simulink model "ElectricVehicleThermalManagementWithHeatPump"  (R2024b)
settings: Solver=VariableStepAuto  StartTime=0.0  StopTime=3600  RelTol=1e-3  AbsTol=1e-3
PreLoadFcn:
  | init_nmpc
InitFcn:
  | init_nmpc
model workspace: external: MATLAB File ElectricVehicleThermalManagementWithHeatPumpParameters.m (data not in the file)
values from neighbouring files (symbols this model uses):
  battery_C1_LUT = [1913.6 12447 30609 ... (first row only)    [ElectricVehicleThermalManagementWithHeatPumpParameters.m]
  battery_capacity_LUT = [280.081 276.25 276.392]    [ElectricVehicleThermalManagementWithHeatPumpParameters.m]
  battery_cell_cp = 795    [ElectricVehicleThermalManagementWithHeatPumpParameters.m]
  battery_cell_mass = 2.5    [ElectricVehicleThermalManagementWithHeatPumpParameters.m]
  battery_Em_LUT = [3.4966 3.5057 3.5148 ... (first row only)    [ElectricVehicleThermalManagementWithHeatPumpParameters.m]
  battery_N_cells = 20    [ElectricVehicleThermalManagementWithHeatPumpParameters.m]
  battery_Qe_init = 0    [ElectricVehicleThermalManagementWithHeatPumpParameters.m]
  battery_R0_LUT = [0.0117 0.0085 0.009 ... (first row only)    [ElectricVehicleThermalManagementWithHeatPumpParameters.m]
  battery_R1_LUT = [0.0109 0.0029 0.0013 ... (first row only)    [ElectricVehicleThermalManagementWithHeatPumpParameters.m]
  battery_SOC_LUT = [0; 0.1; 0.25; 0.5; 0.75; 0.9; 1]    [ElectricVehicleThermalManagementWithHeatPumpParameters.m]
  battery_T_init = -10    [ElectricVehicleThermalManagementWithHeatPumpParameters.m]
  battery_temperature_LUT = [5 20 40]    [ElectricVehicleThermalManagementWithHeatPumpParameters.m]
  cabin_duct_area = 0.04    [ElectricVehicleThermalManagementWithHeatPumpParameters.m]
  cabin_T_init = -10    [ElectricVehicleThermalManagementWithHeatPumpParameters.m]
  chiller_area_primary = 0.43982297150257105    (= 0.439822971503)    [ElectricVehicleThermalManagementWithHeatPumpParameters.m]
  chiller_N_baffles = 3    [ElectricVehicleThermalManagementWithHeatPumpParameters.m]
  chiller_N_tubes = 100    [ElectricVehicleThermalManagementWithHeatPumpParameters.m]
  chiller_tube_D = 0.0035    [ElectricVehicleThermalManagementWithHeatPumpParameters.m]
  chiller_tube_L = 0.4    [ElectricVehicleThermalManagementWithHeatPumpParameters.m]
  chiller_wall_conductivity = 240    [ElectricVehicleThermalManagementWithHeatPumpParameters.m]
  chiller_wall_thickness = 0.0001    [ElectricVehicleThermalManagementWithHeatPumpParameters.m]
  cond_evap_air_area_flow = 0.3906    [ElectricVehicleThermalManagementWithHeatPumpParameters.m]
  cond_evap_air_area_primary = 1.4834999999999998    (= 1.4835)    [ElectricVehicleThermalManagementWithHeatPumpParameters.m]
  cond_evap_W = 0.015    [ElectricVehicleThermalManagementWithHeatPumpParameters.m]
  cond_evap_wall_conductivity = 240    [ElectricVehicleThermalManagementWithHeatPumpParameters.m]
  cond_evap_wall_thickness = 0.0001    [ElectricVehicleThermalManagementWithHeatPumpParameters.m]
  coolant_channel_D = 0.0092    [ElectricVehicleThermalManagementWithHeatPumpParameters.m]
  coolant_pipe_D = 0.019    [ElectricVehicleThermalManagementWithHeatPumpParameters.m]
  coolant_T_init = -10    [ElectricVehicleThermalManagementWithHeatPumpParameters.m]
  coolant_tank_area = 0.0121    [ElectricVehicleThermalManagementWithHeatPumpParameters.m]
  coolant_tank_volume = 1.25    [ElectricVehicleThermalManagementWithHeatPumpParameters.m]
  coolant_valve_D_ratio_max = 0.95    [ElectricVehicleThermalManagementWithHeatPumpParameters.m]
  coolant_valve_D_ratio_min = 0.001    [ElectricVehicleThermalManagementWithHeatPumpParameters.m]
  coolant_valve_displacement = 0.0063    [ElectricVehicleThermalManagementWithHeatPumpParameters.m]
  coolant_valve_S_max = 0.0053    [ElectricVehicleThermalManagementWithHeatPumpParameters.m]
  evaporator_air_area_flow = 0.12    [ElectricVehicleThermalManagementWithHeatPumpParameters.m]
  evaporator_air_area_primary = 0.4323    [ElectricVehicleThermalManagementWithHeatPumpParameters.m]
  evaporator_W = 0.015    [ElectricVehicleThermalManagementWithHeatPumpParameters.m]
  evaporator_wall_conductivity = 240    [ElectricVehicleThermalManagementWithHeatPumpParameters.m]
  evaporator_wall_thickness = 0.0001    [ElectricVehicleThermalManagementWithHeatPumpParameters.m]
  expansion_valve_D_ratio_max = 0.9    [ElectricVehicleThermalManagementWithHeatPumpParameters.m]
  hex_area_primary = 0.070371675440411369    (= 0.0703716754404)    [ElectricVehicleThermalManagementWithHeatPumpParameters.m]
  hex_N_tubes = 64    [ElectricVehicleThermalManagementWithHeatPumpParameters.m]
  hex_tube_D = 0.0035    [ElectricVehicleThermalManagementWithHeatPumpParameters.m]
  hex_wall_conductivity = 240    [ElectricVehicleThermalManagementWithHeatPumpParameters.m]
  hex_wall_thickness = 0.0001    [ElectricVehicleThermalManagementWithHeatPumpParameters.m]
  inner_cond_air_area_flow = 0.1953    [ElectricVehicleThermalManagementWithHeatPumpParameters.m]
  inner_cond_air_area_primary = 0.99520000000000008    (= 0.9952)    [ElectricVehicleThermalManagementWithHeatPumpParameters.m]
  inner_cond_W = 0.02    [ElectricVehicleThermalManagementWithHeatPumpParameters.m]
  inner_cond_wall_conductivity = 240    [ElectricVehicleThermalManagementWithHeatPumpParameters.m]
  inner_cond_wall_thickness = 0.0001    [ElectricVehicleThermalManagementWithHeatPumpParameters.m]
  pump_speed_max = 1000    [ElectricVehicleThermalManagementWithHeatPumpParameters.m]
  radiator_air_area_flow = 0.097499999999999989    (= 0.0975)    [ElectricVehicleThermalManagementWithHeatPumpParameters.m]
  radiator_air_area_primary = 0.43687499999999996    (= 0.436875)    [ElectricVehicleThermalManagementWithHeatPumpParameters.m]
  radiator_W = 0.015    [ElectricVehicleThermalManagementWithHeatPumpParameters.m]
  radiator_wall_conductivity = 240    [ElectricVehicleThermalManagementWithHeatPumpParameters.m]
  radiator_wall_thickness = 0.0001    [ElectricVehicleThermalManagementWithHeatPumpParameters.m]
  refrigerant_p_init = 0.2    [ElectricVehicleThermalManagementWithHeatPumpParameters.m]
  refrigerant_pipe_D = 0.01    [ElectricVehicleThermalManagementWithHeatPumpParameters.m]
  refrigerant_valve_D_ratio_max = 0.95    [ElectricVehicleThermalManagementWithHeatPumpParameters.m]
  refrigerant_valve_displacement = 0.005    [ElectricVehicleThermalManagementWithHeatPumpParameters.m]
libraries: fl_lib x227, nesl_utility x162, SimscapeFluids_lib x30, LiBatteryElements_lib x16, slpidlib x3, SignalEditorBlockLib x1
(part 12 of 13)

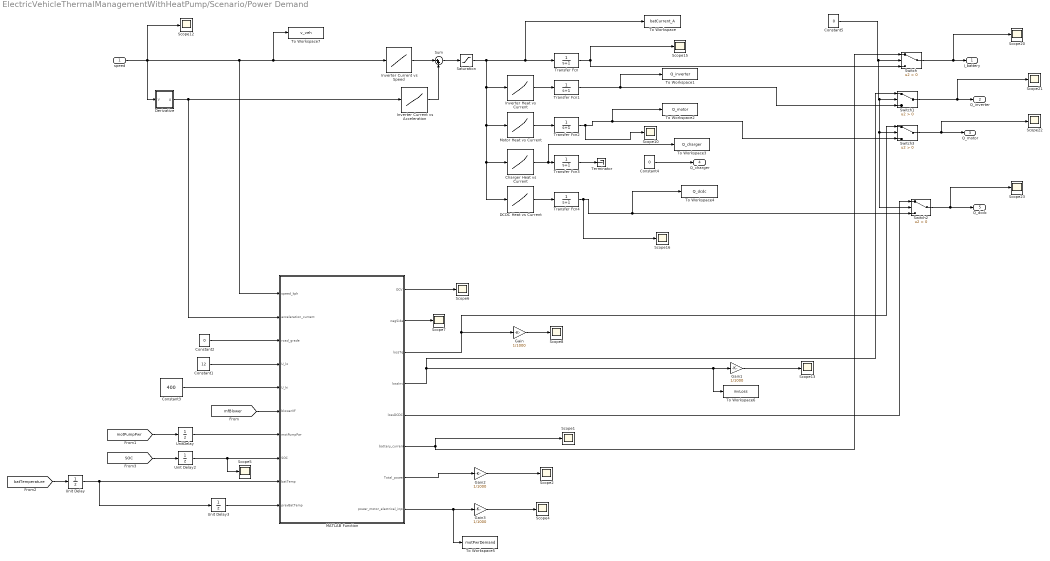
== system ElectricVehicleThermalManagementWithHeatPump/Scenario/Power Demand ==
  speed : Inport
  Charger Heat vs Current : Lookup_n-D  NumberOfTableDimensions=1  BreakpointsForDimension1=[-100 0 25 50 300]  IndexSearchMethod=Linear search  BeginIndexSearchUsingPreviousIndexResult=on  Table=[250 0 40 70 400]  InternalRulePriority=Speed  RndMeth=Simplest
  Constant1 : Constant  Value=12
  Constant2 : Constant  Value=0
  Constant3 : Constant  Value=400
  Constant4 : Constant  Value=0
  Constant5 : Constant  Value=0
  DCDC Heat vs Current : Lookup_n-D  NumberOfTableDimensions=1  BreakpointsForDimension1=[-100 0 25 50 300]  IndexSearchMethod=Linear search  BeginIndexSearchUsingPreviousIndexResult=on  Table=[250 0 40 70 400]  InternalRulePriority=Speed  RndMeth=Simplest
  Derivative : Subsystem  mask(1-st Order Filter Derivative){tau=1}
      mask prompts: tau "Filter time constant [s]"
  Gain{,1..3} (4 alike) : Gain  Gain=1/1000
  Inverter Current vs Acceleration : Lookup_n-D  NumberOfTableDimensions=1  BreakpointsForDimension1=[-10 -8 -5 0 5 8 10]  IndexSearchMethod=Linear search  BeginIndexSearchUsingPreviousIndexResult=on  Table=[200 150 100 0 100 150 200]*0.6  InternalRulePriority=Speed  RndMeth=Simplest
  Inverter Current vs Speed : Lookup_n-D  NumberOfTableDimensions=1  BreakpointsForDimension1=[0 60 80 100 120 140 160 180 200]  IndexSearchMethod=Linear search  BeginIndexSearchUsingPreviousIndexResult=on  Table=[0 10 18 27 45 65 100 120 160]  InternalRulePriority=Speed  RndMeth=Simplest
  Inverter Heat vs Current : Lookup_n-D  NumberOfTableDimensions=1  BreakpointsForDimension1=[-100 0 25 50 300]  IndexSearchMethod=Linear search  BeginIndexSearchUsingPreviousIndexResult=on  Table=[250 0 40 70 400]  InternalRulePriority=Speed  RndMeth=Simplest
  MATLAB Function : MATLAB Function  TreatAsAtomicUnit=on
  Motor Heat vs Current : Lookup_n-D  NumberOfTableDimensions=1  BreakpointsForDimension1=[-150 -70 -26 0 25 50 100 300 600]  IndexSearchMethod=Linear search  BeginIndexSearchUsingPreviousIndexResult=on  Table=[3500 2650 2100 0 400 550 4800 4800 4800]  InternalRulePriority=Speed  RndMeth=Simplest
  Saturation : Saturate  UpperLimit=200  LowerLimit=-inf  ZeroCross=off
  Scope{1..2,4..8,10,12..13,15..16,20..23} (16 alike) : Scope
  Sum : Sum  Inputs=|++
  Switch{,1..3} (4 alike) : Switch  Criteria=u2 > Threshold  SaturateOnIntegerOverflow=off  InputSameDT=off
  Terminator : Terminator
  To Workspace : ToWorkspace  VariableName=batCurrent_A  SampleTime=-1
  To Workspace1 : ToWorkspace  VariableName=Q_inverter  SampleTime=-1
  To Workspace2 : ToWorkspace  VariableName=Q_motor  SampleTime=-1
  To Workspace3 : ToWorkspace  VariableName=Q_charger  SampleTime=-1
  To Workspace4 : ToWorkspace  VariableName=Q_dcdc  SampleTime=-1
  To Workspace5 : ToWorkspace  VariableName=motPwrDemand  SampleTime=-1
  To Workspace6 : ToWorkspace  VariableName=invLoss  SampleTime=-1
  To Workspace7 : ToWorkspace  VariableName=v_veh  SampleTime=-1
  Transfer Fcn{,1..4} (5 alike) : TransferFcn  Denominator=[1 1]
  Unit Delay : UnitDelay  SampleTime=-1  HasFrameUpgradeWarning=on
  Unit Delay2 : UnitDelay  SampleTime=-1  HasFrameUpgradeWarning=on
  Unit Delay3 : UnitDelay  SampleTime=-1  HasFrameUpgradeWarning=on
  UnitDelay : UnitDelay  SampleTime=-1  HasFrameUpgradeWarning=on
  I_battery : Outport
  Q_inverter : Outport  Port=2
  Q_motor : Outport  Port=3
  Q_charger : Outport  Port=4
  Q_dcdc : Outport  Port=5
  wires:
  Derivative/1(A) -> Inverter Current vs Acceleration/1, MATLAB Function/2(acceleration_current)
  speed/1 -> Scope12/1, MATLAB Function/1(speed_kph), To Workspace7/1, Inverter Current vs Speed/1, Derivative/1(V)
  Inverter Current vs Speed/1 -> Sum/1
  Inverter Current vs Acceleration/1 -> Sum/2
  Sum/1 -> Saturation/1
  Inverter Heat vs Current/1 -> Transfer Fcn1/1
  Motor Heat vs Current/1 -> Transfer Fcn2/1
  Charger Heat vs Current/1 -> To Workspace3/1, Transfer Fcn3/1
  Transfer Fcn/1 -> Switch/3, Scope15/1
  Transfer Fcn1/1 -> To Workspace1/1, Switch1/3
  Transfer Fcn2/1 -> Scope10/1, To Workspace2/1, Switch3/3
  DCDC Heat vs Current/1 -> Transfer Fcn4/1
  Transfer Fcn4/1 -> Scope16/1, To Workspace4/1, Switch2/3
  Constant2/1 -> MATLAB Function/3(road_grade)
  MATLAB Function/3(lossTq) -> Switch3/1, Gain/1
  Gain/1 -> Scope8/1
  MATLAB Function/4(lossInv) -> Switch1/1, Gain1/1, To Workspace6/1
  Gain1/1 -> Scope13/1
  MATLAB Function/7(Total_power) -> Gain2/1
  Gain2/1 -> Scope2/1
  Constant1/1 -> MATLAB Function/4(U_lo)
  MATLAB Function/8(power_motor_electrical_input) -> To Workspace5/1, Gain3/1
  Constant3/1 -> MATLAB Function/5(U_hi)
  [mfBlower] -> MATLAB Function/6(blowerVF)
  [batTemperature] -> Unit Delay/1
  [SOC] -> Unit Delay2/1
  Gain3/1 -> Scope4/1
  Saturation/1 -> Inverter Heat vs Current/1, Motor Heat vs Current/1, DCDC Heat vs Current/1, Charger Heat vs Current/1, To Workspace/1, Transfer Fcn/1
  MATLAB Function/6(battery_current) -> Switch/1, Scope1/1
  Switch1/1 -> Scope21/1, Q_inverter/1
  Constant4/1 -> Q_charger/1
  Switch2/1 -> Scope23/1, Q_dcdc/1
  MATLAB Function/5(lossDCDC) -> Switch2/1
  Switch3/1 -> Scope22/1, Q_motor/1
  Constant5/1 -> Switch2/2, Switch3/2, Switch1/2, Switch/2
  Switch/1 -> Scope20/1, I_battery/1
  MATLAB Function/1(OCV) -> Scope6/1
  MATLAB Function/2(negSide) -> Scope7/1
  [motPumpPwr] -> UnitDelay/1
  Unit Delay/1 -> Unit Delay3/1, MATLAB Function/9(batTemp)
  UnitDelay/1 -> MATLAB Function/7(motPumpPwr)
  Unit Delay2/1 -> Scope5/1, MATLAB Function/8(SOC)
  Unit Delay3/1 -> MATLAB Function/10(prevBatTemp)
  Transfer Fcn3/1 -> Terminator/1

== system ElectricVehicleThermalManagementWithHeatPump/Battery/Pack 1/Lithium Cell 1RC ==
  note: Power
      | Losses
  C1 : LiBatteryElements_lib/C_table  C_Table=C1_LUT F  SOC_Table=SOC_LUT  Temp_Table=Temperature_LUT K  v0=0 V
      settings: InternalSimscapePortConfiguration="{\"Bottom\":[],\"Left\":[{\"id\":\"p\",\"label\":\"+\",\"type\":\"foundation.electrical.electrical\"},{\"id\":\"T\",\"label\":\"T\",\"type\":\"input\"},{\"id\":\"SOC\",\"label\":\"SOC\",\"type\":\"input\"}],\"Right\":[{\"id\":\"n\",\"label\":\"-\",\"type\":\"foundation.electrical.electrical\"}],\"Top\":[]}"
  Em_table : LiBatteryElements_lib/Em_table  C_Table=Capacity_LUT hr*A  Em_Table=Em_LUT V  SOC_Table=SOC_LUT  Temp_Table=Temperature_LUT K  Qinit=Qe_init hr*A
      settings: InternalSimscapePortConfiguration="{\"Bottom\":[],\"Left\":[{\"id\":\"p\",\"label\":\"+\",\"type\":\"foundation.electrical.electrical\"},{\"id\":\"C\",\"label\":\"C\",\"type\":\"output\"},{\"id\":\"SOC\",\"label\":\"SOC\",\"type\":\"output\"}],\"Right\":[{\"id\":\"n\",\"label\":\"-\",\"type\":\"foundation.electrical.electrical\"},{\"id\":\"T\",\"label\":\"T\",\"type\":\"input\"}],\"Top\":[]}"
  PS-Simulink Converter : nesl_utility/PS-Simulink Converter  PhysicalDomain=network_engine_domain  SubClassName=ps_output  LeftPortType=input  RightPortType=output  PseudoPeriodic=off  Frequencies=[]  VectorFormat=inherit  Unit=inherit  AffineConversion=off
  PS-Simulink Converter1 : nesl_utility/PS-Simulink Converter  PhysicalDomain=network_engine_domain  SubClassName=ps_output  LeftPortType=input  RightPortType=output  PseudoPeriodic=off  Frequencies=[]  VectorFormat=inherit  Unit=inherit  AffineConversion=off
  Power Sum : fl_lib/Physical Signals/Functions/PS Add
  R0 : LiBatteryElements_lib/R_table  R_Table=R0_LUT Ohm  SOC_Table=SOC_LUT  Temp_Table=Temperature_LUT K
      settings: InternalSimscapePortConfiguration="{\"Bottom\":[],\"Left\":[{\"id\":\"p\",\"label\":\"+\",\"type\":\"foundation.electrical.electrical\"},{\"id\":\"T\",\"label\":\"T\",\"type\":\"input\"},{\"id\":\"SOC\",\"label\":\"SOC\",\"type\":\"input\"}],\"Right\":[{\"id\":\"n\",\"label\":\"-\",\"type\":\"foundation.electrical.electrical\"},{\"id\":\"pow\",\"label\":\"POW\",\"type\":\"output\"}],\"Top\":[]}"
  R1 : LiBatteryElements_lib/R_table  R_Table=R1_LUT Ohm  SOC_Table=SOC_LUT  Temp_Table=Temperature_LUT K
      settings: InternalSimscapePortConfiguration="{\"Bottom\":[],\"Left\":[{\"id\":\"p\",\"label\":\"+\",\"type\":\"foundation.electrical.electrical\"},{\"id\":\"T\",\"label\":\"T\",\"type\":\"input\"},{\"id\":\"SOC\",\"label\":\"SOC\",\"type\":\"input\"}],\"Right\":[{\"id\":\"n\",\"label\":\"-\",\"type\":\"foundation.electrical.electrical\"},{\"id\":\"pow\",\"label\":\"POW\",\"type\":\"output\"}],\"Top\":[]}"
  Scope : Scope
  Scope1 : Scope
  To Workspace : ToWorkspace  VariableName=soc_meas  SampleTime=-1
  P : PMIOPort  Side=Left
  + : PMIOPort  Port=2  Side=Left
  T : PMIOPort  Port=3  Side=Right
  - : PMIOPort  Port=4  Side=Right
  tag scope: SOC=global
  wires:
  PS-Simulink Converter/1 -> To Workspace/1, [SOC], Scope/1
  PS-Simulink Converter1/1 -> Scope1/1
  connections:
  R1/RConn2 -- Power Sum/LConn1
  Power Sum/LConn2 -- R0/RConn2
  P/RConn1 -- Power Sum/RConn1
  +/RConn1 -- R0/RConn1
  T/RConn1 -- Em_table/RConn2 -- R0/LConn2 -- C1/LConn2 -- R1/LConn2
  Em_table/LConn1 -- C1/LConn1 -- R1/LConn1
  C1/RConn1 -- R1/RConn1 -- R0/LConn1
  Em_table/RConn1 -- -/RConn1
  C1/LConn3 -- PS-Simulink Converter/LConn1 -- R0/LConn3 -- Em_table/LConn3 -- R1/LConn3
  PS-Simulink Converter1/LConn1 -- Em_table/LConn2

== system ElectricVehicleThermalManagementWithHeatPump/Battery/Pack 1/Thermal Model ==
  Battery Thermal Mass : fl_lib/Thermal/Thermal Elements/Thermal Mass  mass_type=foundation.enum.constant_variable.constant  mass=cell_mass*Ncells kg  sp_heat=cell_Cp_heat J/kg/K  mass_min=1e-6 kg  num_ports=foundation.enum.numPorts2.one  m_specify=off  m_priority=High  m=1 kg  m_nominal_specify=off  m_nominal_value=1  m_nominal_unit=kg  T_specify=on  T_priority=High  T=T_init K  T_nominal_specify=off  T_nominal_value=1  T_nominal_unit=K  Q_specify=off  Q_priority=None  Q=0 W  Q_nominal_specify=off  Q_nominal_value=1  Q_nominal_unit=W
  Controlled Heat Flow Rate Source : fl_lib/Thermal/Thermal Sources/Controlled Heat Flow Rate Source
  Temperature Sensor : fl_lib/Thermal/Thermal Sensors/Temperature Sensor  temperature_measure=foundation.enum.MeasurementReference.difference
  Thermal Reference : fl_lib/Thermal/Thermal Elements/Thermal Reference
  Thermal Reference2 : fl_lib/Thermal/Thermal Elements/Thermal Reference
  H : PMIOPort  Side=Left
  Pxn : PMIOPort  Port=2  Side=Left
  T : PMIOPort  Port=3  Side=Right
  connections:
  H/RConn1 -- Controlled Heat Flow Rate Source/LConn1 -- Battery Thermal Mass/LConn1 -- Temperature Sensor/LConn1
  Pxn/RConn1 -- Controlled Heat Flow Rate Source/RConn1
  Controlled Heat Flow Rate Source/RConn2 -- Thermal Reference2/LConn1
  Thermal Reference/LConn1 -- Temperature Sensor/RConn1
  T/RConn1 -- Temperature Sensor/RConn2

== system ElectricVehicleThermalManagementWithHeatPump/Battery/Pack 2/Lithium Cell 1RC ==
  note: Power
      | Losses
  C1 : LiBatteryElements_lib/C_table  C_Table=C1_LUT F  SOC_Table=SOC_LUT  Temp_Table=Temperature_LUT K  v0=0 V
      settings: InternalSimscapePortConfiguration="{\"Bottom\":[],\"Left\":[{\"id\":\"p\",\"label\":\"+\",\"type\":\"foundation.electrical.electrical\"},{\"id\":\"T\",\"label\":\"T\",\"type\":\"input\"},{\"id\":\"SOC\",\"label\":\"SOC\",\"type\":\"input\"}],\"Right\":[{\"id\":\"n\",\"label\":\"-\",\"type\":\"foundation.electrical.electrical\"}],\"Top\":[]}"
  Em_table : LiBatteryElements_lib/Em_table  C_Table=Capacity_LUT hr*A  Em_Table=Em_LUT V  SOC_Table=SOC_LUT  Temp_Table=Temperature_LUT K  Qinit=Qe_init hr*A
      settings: InternalSimscapePortConfiguration="{\"Bottom\":[],\"Left\":[{\"id\":\"p\",\"label\":\"+\",\"type\":\"foundation.electrical.electrical\"},{\"id\":\"C\",\"label\":\"C\",\"type\":\"output\"},{\"id\":\"SOC\",\"label\":\"SOC\",\"type\":\"output\"}],\"Right\":[{\"id\":\"n\",\"label\":\"-\",\"type\":\"foundation.electrical.electrical\"},{\"id\":\"T\",\"label\":\"T\",\"type\":\"input\"}],\"Top\":[]}"
  Power Sum : fl_lib/Physical Signals/Functions/PS Add
  R0 : LiBatteryElements_lib/R_table  R_Table=R0_LUT Ohm  SOC_Table=SOC_LUT  Temp_Table=Temperature_LUT K
      settings: InternalSimscapePortConfiguration="{\"Bottom\":[],\"Left\":[{\"id\":\"p\",\"label\":\"+\",\"type\":\"foundation.electrical.electrical\"},{\"id\":\"T\",\"label\":\"T\",\"type\":\"input\"},{\"id\":\"SOC\",\"label\":\"SOC\",\"type\":\"input\"}],\"Right\":[{\"id\":\"n\",\"label\":\"-\",\"type\":\"foundation.electrical.electrical\"},{\"id\":\"pow\",\"label\":\"POW\",\"type\":\"output\"}],\"Top\":[]}"
  R1 : LiBatteryElements_lib/R_table  R_Table=R1_LUT Ohm  SOC_Table=SOC_LUT  Temp_Table=Temperature_LUT K
      settings: InternalSimscapePortConfiguration="{\"Bottom\":[],\"Left\":[{\"id\":\"p\",\"label\":\"+\",\"type\":\"foundation.electrical.electrical\"},{\"id\":\"T\",\"label\":\"T\",\"type\":\"input\"},{\"id\":\"SOC\",\"label\":\"SOC\",\"type\":\"input\"}],\"Right\":[{\"id\":\"n\",\"label\":\"-\",\"type\":\"foundation.electrical.electrical\"},{\"id\":\"pow\",\"label\":\"POW\",\"type\":\"output\"}],\"Top\":[]}"
  P : PMIOPort  Side=Left
  + : PMIOPort  Port=2  Side=Left
  T : PMIOPort  Port=3  Side=Right
  - : PMIOPort  Port=4  Side=Right
  connections:
  R1/RConn2 -- Power Sum/LConn1
  Power Sum/LConn2 -- R0/RConn2
  P/RConn1 -- Power Sum/RConn1
  +/RConn1 -- R0/RConn1
  T/RConn1 -- Em_table/RConn2 -- R0/LConn2 -- C1/LConn2 -- R1/LConn2
  Em_table/LConn1 -- C1/LConn1 -- R1/LConn1
  C1/RConn1 -- R1/RConn1 -- R0/LConn1
  Em_table/RConn1 -- -/RConn1
  C1/LConn3 -- Em_table/LConn3 -- R1/LConn3 -- R0/LConn3

== system ElectricVehicleThermalManagementWithHeatPump/Battery/Pack 2/Thermal Model ==
  Battery Thermal Mass : fl_lib/Thermal/Thermal Elements/Thermal Mass  mass_type=foundation.enum.constant_variable.constant  mass=cell_mass*Ncells kg  sp_heat=cell_Cp_heat J/kg/K  mass_min=1e-6 kg  num_ports=foundation.enum.numPorts2.one  m_specify=off  m_priority=High  m=1 kg  m_nominal_specify=off  m_nominal_value=1  m_nominal_unit=kg  T_specify=on  T_priority=High  T=T_init K  T_nominal_specify=off  T_nominal_value=1  T_nominal_unit=K  Q_specify=off  Q_priority=None  Q=0 W  Q_nominal_specify=off  Q_nominal_value=1  Q_nominal_unit=W
  Controlled Heat Flow Rate Source : fl_lib/Thermal/Thermal Sources/Controlled Heat Flow Rate Source
  Temperature Sensor : fl_lib/Thermal/Thermal Sensors/Temperature Sensor  temperature_measure=foundation.enum.MeasurementReference.difference
  Thermal Reference : fl_lib/Thermal/Thermal Elements/Thermal Reference
  Thermal Reference2 : fl_lib/Thermal/Thermal Elements/Thermal Reference
  H : PMIOPort  Side=Left
  Pxn : PMIOPort  Port=2  Side=Left
  T : PMIOPort  Port=3  Side=Right
  connections:
  H/RConn1 -- Controlled Heat Flow Rate Source/LConn1 -- Battery Thermal Mass/LConn1 -- Temperature Sensor/LConn1
  Pxn/RConn1 -- Controlled Heat Flow Rate Source/RConn1
  Controlled Heat Flow Rate Source/RConn2 -- Thermal Reference2/LConn1
  Thermal Reference/LConn1 -- Temperature Sensor/RConn1
  T/RConn1 -- Temperature Sensor/RConn2

== system ElectricVehicleThermalManagementWithHeatPump/Battery/Pack 3/Lithium Cell 1RC ==
  note: Power
      | Losses
  C1 : LiBatteryElements_lib/C_table  C_Table=C1_LUT F  SOC_Table=SOC_LUT  Temp_Table=Temperature_LUT K  v0=0 V
      settings: InternalSimscapePortConfiguration="{\"Bottom\":[],\"Left\":[{\"id\":\"p\",\"label\":\"+\",\"type\":\"foundation.electrical.electrical\"},{\"id\":\"T\",\"label\":\"T\",\"type\":\"input\"},{\"id\":\"SOC\",\"label\":\"SOC\",\"type\":\"input\"}],\"Right\":[{\"id\":\"n\",\"label\":\"-\",\"type\":\"foundation.electrical.electrical\"}],\"Top\":[]}"
  Em_table : LiBatteryElements_lib/Em_table  C_Table=Capacity_LUT hr*A  Em_Table=Em_LUT V  SOC_Table=SOC_LUT  Temp_Table=Temperature_LUT K  Qinit=Qe_init hr*A
      settings: InternalSimscapePortConfiguration="{\"Bottom\":[],\"Left\":[{\"id\":\"p\",\"label\":\"+\",\"type\":\"foundation.electrical.electrical\"},{\"id\":\"C\",\"label\":\"C\",\"type\":\"output\"},{\"id\":\"SOC\",\"label\":\"SOC\",\"type\":\"output\"}],\"Right\":[{\"id\":\"n\",\"label\":\"-\",\"type\":\"foundation.electrical.electrical\"},{\"id\":\"T\",\"label\":\"T\",\"type\":\"input\"}],\"Top\":[]}"
  Power Sum : fl_lib/Physical Signals/Functions/PS Add
  R0 : LiBatteryElements_lib/R_table  R_Table=R0_LUT Ohm  SOC_Table=SOC_LUT  Temp_Table=Temperature_LUT K
      settings: InternalSimscapePortConfiguration="{\"Bottom\":[],\"Left\":[{\"id\":\"p\",\"label\":\"+\",\"type\":\"foundation.electrical.electrical\"},{\"id\":\"T\",\"label\":\"T\",\"type\":\"input\"},{\"id\":\"SOC\",\"label\":\"SOC\",\"type\":\"input\"}],\"Right\":[{\"id\":\"n\",\"label\":\"-\",\"type\":\"foundation.electrical.electrical\"},{\"id\":\"pow\",\"label\":\"POW\",\"type\":\"output\"}],\"Top\":[]}"
  R1 : LiBatteryElements_lib/R_table  R_Table=R1_LUT Ohm  SOC_Table=SOC_LUT  Temp_Table=Temperature_LUT K
      settings: InternalSimscapePortConfiguration="{\"Bottom\":[],\"Left\":[{\"id\":\"p\",\"label\":\"+\",\"type\":\"foundation.electrical.electrical\"},{\"id\":\"T\",\"label\":\"T\",\"type\":\"input\"},{\"id\":\"SOC\",\"label\":\"SOC\",\"type\":\"input\"}],\"Right\":[{\"id\":\"n\",\"label\":\"-\",\"type\":\"foundation.electrical.electrical\"},{\"id\":\"pow\",\"label\":\"POW\",\"type\":\"output\"}],\"Top\":[]}"
  P : PMIOPort  Side=Left
  + : PMIOPort  Port=2  Side=Left
  T : PMIOPort  Port=3  Side=Right
  - : PMIOPort  Port=4  Side=Right
  connections:
  R0/LConn3 -- R1/LConn3 -- Em_table/LConn3 -- C1/LConn3
  Em_table/RConn1 -- -/RConn1
  R0/LConn1 -- R1/RConn1 -- C1/RConn1
  R1/LConn1 -- C1/LConn1 -- Em_table/LConn1
  R1/LConn2 -- C1/LConn2 -- R0/LConn2 -- Em_table/RConn2 -- T/RConn1
  +/RConn1 -- R0/RConn1
  P/RConn1 -- Power Sum/RConn1
  Power Sum/LConn2 -- R0/RConn2
  R1/RConn2 -- Power Sum/LConn1

== system ElectricVehicleThermalManagementWithHeatPump/Battery/Pack 3/Thermal Model ==
  Battery Thermal Mass : fl_lib/Thermal/Thermal Elements/Thermal Mass  mass_type=foundation.enum.constant_variable.constant  mass=cell_mass*Ncells kg  sp_heat=cell_Cp_heat J/kg/K  mass_min=1e-6 kg  num_ports=foundation.enum.numPorts2.one  m_specify=off  m_priority=High  m=1 kg  m_nominal_specify=off  m_nominal_value=1  m_nominal_unit=kg  T_specify=on  T_priority=High  T=T_init K  T_nominal_specify=off  T_nominal_value=1  T_nominal_unit=K  Q_specify=off  Q_priority=None  Q=0 W  Q_nominal_specify=off  Q_nominal_value=1  Q_nominal_unit=W
  Controlled Heat Flow Rate Source : fl_lib/Thermal/Thermal Sources/Controlled Heat Flow Rate Source
  Temperature Sensor : fl_lib/Thermal/Thermal Sensors/Temperature Sensor  temperature_measure=foundation.enum.MeasurementReference.difference
  Thermal Reference : fl_lib/Thermal/Thermal Elements/Thermal Reference
  Thermal Reference2 : fl_lib/Thermal/Thermal Elements/Thermal Reference
  H : PMIOPort  Side=Left
  Pxn : PMIOPort  Port=2  Side=Left
  T : PMIOPort  Port=3  Side=Right
  connections:
  T/RConn1 -- Temperature Sensor/RConn2
  Thermal Reference/LConn1 -- Temperature Sensor/RConn1
  Controlled Heat Flow Rate Source/RConn2 -- Thermal Reference2/LConn1
  Pxn/RConn1 -- Controlled Heat Flow Rate Source/RConn1
  Temperature Sensor/LConn1 -- Battery Thermal Mass/LConn1 -- Controlled Heat Flow Rate Source/LConn1 -- H/RConn1

== system ElectricVehicleThermalManagementWithHeatPump/Battery/Pack 4/Lithium Cell 1RC ==
  note: Power
      | Losses
  C1 : LiBatteryElements_lib/C_table  C_Table=C1_LUT F  SOC_Table=SOC_LUT  Temp_Table=Temperature_LUT K  v0=0 V
      settings: InternalSimscapePortConfiguration="{\"Bottom\":[],\"Left\":[{\"id\":\"p\",\"label\":\"+\",\"type\":\"foundation.electrical.electrical\"},{\"id\":\"T\",\"label\":\"T\",\"type\":\"input\"},{\"id\":\"SOC\",\"label\":\"SOC\",\"type\":\"input\"}],\"Right\":[{\"id\":\"n\",\"label\":\"-\",\"type\":\"foundation.electrical.electrical\"}],\"Top\":[]}"
  Em_table : LiBatteryElements_lib/Em_table  C_Table=Capacity_LUT hr*A  Em_Table=Em_LUT V  SOC_Table=SOC_LUT  Temp_Table=Temperature_LUT K  Qinit=Qe_init hr*A
      settings: InternalSimscapePortConfiguration="{\"Bottom\":[],\"Left\":[{\"id\":\"p\",\"label\":\"+\",\"type\":\"foundation.electrical.electrical\"},{\"id\":\"C\",\"label\":\"C\",\"type\":\"output\"},{\"id\":\"SOC\",\"label\":\"SOC\",\"type\":\"output\"}],\"Right\":[{\"id\":\"n\",\"label\":\"-\",\"type\":\"foundation.electrical.electrical\"},{\"id\":\"T\",\"label\":\"T\",\"type\":\"input\"}],\"Top\":[]}"
  Power Sum : fl_lib/Physical Signals/Functions/PS Add
  R0 : LiBatteryElements_lib/R_table  R_Table=R0_LUT Ohm  SOC_Table=SOC_LUT  Temp_Table=Temperature_LUT K
      settings: InternalSimscapePortConfiguration="{\"Bottom\":[],\"Left\":[{\"id\":\"p\",\"label\":\"+\",\"type\":\"foundation.electrical.electrical\"},{\"id\":\"T\",\"label\":\"T\",\"type\":\"input\"},{\"id\":\"SOC\",\"label\":\"SOC\",\"type\":\"input\"}],\"Right\":[{\"id\":\"n\",\"label\":\"-\",\"type\":\"foundation.electrical.electrical\"},{\"id\":\"pow\",\"label\":\"POW\",\"type\":\"output\"}],\"Top\":[]}"
  R1 : LiBatteryElements_lib/R_table  R_Table=R1_LUT Ohm  SOC_Table=SOC_LUT  Temp_Table=Temperature_LUT K
      settings: InternalSimscapePortConfiguration="{\"Bottom\":[],\"Left\":[{\"id\":\"p\",\"label\":\"+\",\"type\":\"foundation.electrical.electrical\"},{\"id\":\"T\",\"label\":\"T\",\"type\":\"input\"},{\"id\":\"SOC\",\"label\":\"SOC\",\"type\":\"input\"}],\"Right\":[{\"id\":\"n\",\"label\":\"-\",\"type\":\"foundation.electrical.electrical\"},{\"id\":\"pow\",\"label\":\"POW\",\"type\":\"output\"}],\"Top\":[]}"
  P : PMIOPort  Side=Left
  + : PMIOPort  Port=2  Side=Left
  T : PMIOPort  Port=3  Side=Right
  - : PMIOPort  Port=4  Side=Right
  connections:
  R1/RConn2 -- Power Sum/LConn1
  Power Sum/LConn2 -- R0/RConn2
  P/RConn1 -- Power Sum/RConn1
  +/RConn1 -- R0/RConn1
  T/RConn1 -- Em_table/RConn2 -- R0/LConn2 -- C1/LConn2 -- R1/LConn2
  Em_table/LConn1 -- C1/LConn1 -- R1/LConn1
  C1/RConn1 -- R1/RConn1 -- R0/LConn1
  Em_table/RConn1 -- -/RConn1
  C1/LConn3 -- Em_table/LConn3 -- R1/LConn3 -- R0/LConn3

== system ElectricVehicleThermalManagementWithHeatPump/Battery/Pack 4/Thermal Model ==
  Battery Thermal Mass : fl_lib/Thermal/Thermal Elements/Thermal Mass  mass_type=foundation.enum.constant_variable.constant  mass=cell_mass*Ncells kg  sp_heat=cell_Cp_heat J/kg/K  mass_min=1e-6 kg  num_ports=foundation.enum.numPorts2.one  m_specify=off  m_priority=High  m=1 kg  m_nominal_specify=off  m_nominal_value=1  m_nominal_unit=kg  T_specify=on  T_priority=High  T=T_init K  T_nominal_specify=off  T_nominal_value=1  T_nominal_unit=K  Q_specify=off  Q_priority=None  Q=0 W  Q_nominal_specify=off  Q_nominal_value=1  Q_nominal_unit=W
  Controlled Heat Flow Rate Source : fl_lib/Thermal/Thermal Sources/Controlled Heat Flow Rate Source
  Temperature Sensor : fl_lib/Thermal/Thermal Sensors/Temperature Sensor  temperature_measure=foundation.enum.MeasurementReference.difference
  Thermal Reference : fl_lib/Thermal/Thermal Elements/Thermal Reference
  Thermal Reference2 : fl_lib/Thermal/Thermal Elements/Thermal Reference
  H : PMIOPort  Side=Left
  Pxn : PMIOPort  Port=2  Side=Left
  T : PMIOPort  Port=3  Side=Right
  connections:
  H/RConn1 -- Controlled Heat Flow Rate Source/LConn1 -- Battery Thermal Mass/LConn1 -- Temperature Sensor/LConn1
  Pxn/RConn1 -- Controlled Heat Flow Rate Source/RConn1
  Controlled Heat Flow Rate Source/RConn2 -- Thermal Reference2/LConn1
  Thermal Reference/LConn1 -- Temperature Sensor/RConn1
  T/RConn1 -- Temperature Sensor/RConn2

== system ElectricVehicleThermalManagementWithHeatPump/Controls/Cabin Air Control/Blower Control ==
  T_cabin : Inport
  T_cabin_sp : Inport  Port=2
  T_env : Inport  Port=3
  PID Controller : slpidlib/PID Controller  Controller=PI  Form=Parallel  TimeDomain=Continuous-time  UseExternalTs=off  SampleTime=-1  IntegratorMethod=Forward Euler  FilterMethod=Forward Euler  ControllerParametersSource=internal  P=0.5  I=2e-3  UseKiTs=off  D=0  UseExternalDerivativeSource=off  N=100  UseFilter=on  TunerSelectOption=Transfer Function Based (PID Tuner App)  ZeroCross=off  InitialConditionSource=internal  InitialConditionForIntegrator=0  InitialConditionForFilter=0  DifferentiatorICPrevScaledInput=0  ExternalReset=either  TrackingMode=off  Kt=1  LimitOutput=on  SatLimitsSource=internal  UpperSaturationLimit=1  LowerSaturationLimit=0  LinearizeAsGain=on  AntiWindupMode=back-calculation  Kb=1  LimitIntegrator=off  UpperIntegratorSaturationLimit=inf  LowerIntegratorSaturationLimit=-inf  POutMin=[]  POutMax=[]  IOutMin=[]  IOutMax=[]  DOutMin=[]  DOutMax=[]  NOutMin=[]  NOutMax=[]  SumOutMin=[]  SumOutMax=[]  SaturationOutMin=[]  SaturationOutMax=[]  PParamMin=[]  PParamMax=[]  IParamMin=[]  IParamMax=[]  DParamMin=[]  DParamMax=[]  NParamMin=[]  NParamMax=[]  KbParamMin=[]  KbParamMax=[]  KtParamMin=[]  KtParamMax=[]  KbOutMin=[]  KbOutMax=[]  KtOutMin=[]  KtOutMax=[]  IntegratorOutMin=[]  IntegratorOutMax=[]  FilterOutMin=[]  FilterOutMax=[]  SumI1OutMin=[]  SumI1OutMax=[]  SumI2OutMin=[]  SumI2OutMax=[]  SumI3OutMin=[]  SumI3OutMax=[]  SumI4OutMin=[]  SumI4OutMax=[]  SumDOutMin=[]  SumDOutMax=[]  DifferentiatorOutMin=[]  DifferentiatorOutMax=[]  FilterDiffOutCoefMin=[]  FilterDiffOutCoefMax=[]  ReciprocalOutMin=[]  ReciprocalOutMax=[]  SumDenOutMin=[]  SumDenOutMax=[]  SumNumOutMin=[]  SumNumOutMax=[]  DivideOutMin=[]  DivideOutMax=[]  UdiffTsProdOutMin=[]  UdiffTsProdOutMax=[]  NTsProdOutMin=[]  NTsProdOutMax=[]  UintegralTsProdOutMin=[]  UintegralTsProdOutMax=[]  UngainTsProdOutMin=[]  UngainTsProdOutMax=[]  ClampingZeroOutDataTypeStr=Inherit: Inherit via back propagation  ClampingZeroOutMin=[]  ClampingZeroOutMax=[]  FilterDenConstantOutDataTypeStr=Inherit: Inherit via back propagation  FilterDenConstantOutMin=[]  FilterDenConstantOutMax=[]  PCopyOutDataTypeStr=Inherit: Inherit via back propagation  PCopyOutMin=[]  PCopyOutMax=[]  NCopyOutDataTypeStr=Inherit: Inherit via back propagation  NCopyOutMin=[]  NCopyOutMax=[]  IntegratorContinuousStateAttributes=''  IntegratorStateMustResolveToSignalObject=off  IntegratorRTWStateStorageClass=Auto  FilterContinuousStateAttributes=''  FilterStateMustResolveToSignalObject=off  FilterRTWStateStorageClass=Auto  ParallelPVariant=InternalParameters  IdealPVariant=Disabled  IVariant=InternalParameters  DVariant=Disabled  IntegratorVariant=Continuous  SatVariant=Enabled  AWVariant=BackCalculation  PCopyVariant=Disabled  TRVariant=Disabled  FdbkBlocksVariant=Forward  IdealPFdbkVariant=Disabled  SatFdbkVariant=Disabled  DerivativeFilterVariant=Disabled  NVariant=Disabled  NCopyVariant=Disabled_SignalSpec  FilterICVariant=Disabled  IntegratorICVariant=InternalICs  ExternalResetVariant=ExternalReset  TRSumVariant=Passthrough  SumFdbkVariant=Disabled  SumVariant=Sum_PI  TsampFilterVariant=InternalTs  TsampNgainVariant=Passthrough  TsampIntegralVariant=Disabled_SignalSpec  ExternalSaturationOutDataTypeStr=Inherit: Same as second input  DerivativeSourceVariant=Disabled  PreIntVariant=InternalPreInt
  Product : Product
  Sign : Signum
  Sum : Sum  Inputs=-+|
  Sum1 : Sum  Inputs=-+|
  cmd_blower : Outport
  wires:
  T_cabin/1 -> Sum/2
  Sum/1 -> Product/1
  PID Controller/1 -> cmd_blower/1
  T_env/1 -> Sum1/2
  Sign/1 -> PID Controller/2, Product/2
  Product/1 -> PID Controller/1
  Sum1/1 -> Sign/1
  T_cabin_sp/1 -> Sum1/1, Sum/1

== system ElectricVehicleThermalManagementWithHeatPump/Controls/Cabin Air Control/Comfort ==
  T_cabin : Inport
  T_desired : Inport  Port=2
  T_env : Inport  Port=3
  Bias : Bias  Bias=-21  SaturateOnIntegerOverflow=off
  Correction : Lookup_n-D  NumberOfTableDimensions=1  BreakpointsForDimension1=[-100 -10 0 10 100]  BeginIndexSearchUsingPreviousIndexResult=on  Table=[20 15 0 -15 -20]  InternalRulePriority=Speed  RndMeth=Simplest
  Gain : Gain
  Recirculation : Lookup_n-D  NumberOfTableDimensions=1  BreakpointsForDimension1=|  BeginIndexSearchUsingPreviousIndexResult=on  Table=[1 0.9 0.5 0 0.2 0.9 1]  ExtrapMethod=Clip  InternalRulePriority=Speed  RndMeth=Simplest
      | [-20
      | -10
      | 0
      | 20
      | 30
      | 40
      | 50]
  Scope : Scope
  Sum : Sum  Inputs=|+-
  Sum1 : Sum  Inputs=++|
  Sum2 : Sum  Inputs=++|
  Target Cabin Temperature : Lookup_n-D  NumberOfTableDimensions=1  BreakpointsForDimension1=|  BeginIndexSearchUsingPreviousIndexResult=on  Table=[25 24 23 22 21 20 19 19]  InternalRulePriority=Speed  RndMeth=Simplest
      | [-40
      | -20
      | 0
      | 20
      | 30
      | 40
      | 50
      | 80]
  Target Vent Temperature : Lookup_n-D  NumberOfTableDimensions=1  BreakpointsForDimension1=|  BeginIndexSearchUsingPreviousIndexResult=on  Table=[65 52 36 21 14 7 3 3]  InternalRulePriority=Speed  RndMeth=Simplest
      | [-40
      | -20
      | 0
      | 20
      | 30
      | 40
      | 50
      | 80]
  T_cabin_sp : Outport
  T_vent_sp : Outport  Port=2
  cmd_recirc : Outport  Port=3
  wires:
  T_env/1 -> Recirculation/1, Target Vent Temperature/1, Target Cabin Temperature/1
  T_cabin/1 -> Sum/1
  Sum/1 -> Gain/1
  Gain/1 -> Correction/1
  Sum1/1 -> T_vent_sp/1
  Correction/1 -> Sum1/1
  Target Vent Temperature/1 -> Sum1/2
  Recirculation/1 -> cmd_recirc/1
  Sum2/1 -> Sum/2
  Target Cabin Temperature/1 -> Sum2/2
  T_desired/1 -> T_cabin_sp/1, Bias/1
  Bias/1 -> Sum2/1

== system ElectricVehicleThermalManagementWithHeatPump/Controls/Coolant Loop Control/Battery Pump Control ==
  cmd_motor_pump : Inport
  T_battery : Inport  Port=2
  cmd_parallel_serial : Inport  Port=3
  Relay : Relay  OnSwitchValue=45  OffSwitchValue=40  OffOutputValue=0.5
  Switch : Switch  Criteria=u2 > Threshold  Threshold=0.5  SaturateOnIntegerOverflow=off  InputSameDT=off
  cmd_battery_pump : Outport
  wires:
  T_battery/1 -> Relay/1
  cmd_parallel_serial/1 -> Switch/2
  Switch/1 -> cmd_battery_pump/1
  Relay/1 -> Switch/3
  cmd_motor_pump/1 -> Switch/1

== system ElectricVehicleThermalManagementWithHeatPump/Controls/Coolant Loop Control/Motor Pump Control ==
  T_motor : Inport
  1-D Lookup Table : Lookup_n-D  NumberOfTableDimensions=1  BreakpointsForDimension1=[-50 45 48 52 58 60 75 130]  IndexSearchMethod=Linear search  BeginIndexSearchUsingPreviousIndexResult=on  Table=[0 0 0.1 0.3 0.5 0.7 1 1]  ExtrapMethod=Clip  InternalRulePriority=Speed  RndMeth=Simplest
  Saturation : Saturate  UpperLimit=1  LowerLimit=0.3  ZeroCross=off
  cmd_motor_pump : Outport
  wires:
  T_motor/1 -> 1-D Lookup Table/1
  1-D Lookup Table/1 -> Saturation/1
  Saturation/1 -> cmd_motor_pump/1

== system ElectricVehicleThermalManagementWithHeatPump/Controls/Coolant Loop Control/Parallel-Serial Mode ==
  note: 0 = Parallel mode
      |
      | 1 = Serial mode
  thermal_mode : Inport
  T_env : Inport  Port=2
  T_coolant_inverter_out : Inport  Port=3
  Constant : Constant
  MinMax : MinMax  Function=max  Inputs=2  ZeroCross=off
  Relay : Relay  OnSwitchValue=35  OffSwitchValue=30  OnOutputValue=0  OffOutputValue=1
  Switch : Switch  Criteria=u2 > Threshold  Threshold=1  SaturateOnIntegerOverflow=off  InputSameDT=off
  cmd_parallel_serial : Outport
  wires:
  T_env/1 -> MinMax/1
  T_coolant_inverter_out/1 -> MinMax/2
  MinMax/1 -> Relay/1
  Switch/1 -> cmd_parallel_serial/1
  thermal_mode/1 -> Switch/2
  Constant/1 -> Switch/1
  Relay/1 -> Switch/3

== system ElectricVehicleThermalManagementWithHeatPump/Controls/Fan Control/Condenser Requirement ==
  p_cond : Inport
  T_env : Inport  Port=2
  1-D Lookup Table : Lookup_n-D  NumberOfTableDimensions=1  BreakpointsForDimension1=[0 20 30 40 50]  IndexSearchMethod=Linear search  BeginIndexSearchUsingPreviousIndexResult=on  Table=[2.0 2.0 1.8 1.5 1.3]  InternalRulePriority=Speed  RndMeth=Simplest
  1-D Lookup Table1 : Lookup_n-D  NumberOfTableDimensions=1  BreakpointsForDimension1=[0 20 30 40 50]  IndexSearchMethod=Linear search  BeginIndexSearchUsingPreviousIndexResult=on  Table=[1.4 1.4 1.3 1.2 1.1]  InternalRulePriority=Speed  RndMeth=Simplest
  1-D Lookup Table2 : Lookup_n-D  NumberOfTableDimensions=1  BreakpointsForDimension1=[0 20 30 40 50]  IndexSearchMethod=Linear search  BeginIndexSearchUsingPreviousIndexResult=on  Table=[0.8 0.8 0.8 0.8 0.8]  InternalRulePriority=Speed  RndMeth=Simplest
  Bias : Bias  Bias=0.4  SaturateOnIntegerOverflow=off
  Bias1 : Bias  Bias=0.4  SaturateOnIntegerOverflow=off
  Bias2 : Bias  Bias=0.3  SaturateOnIntegerOverflow=off
  Relay Level 1 : Subsystem
  Relay Level 2 : Subsystem
  Relay Level 3 : Subsystem
  Scope : Scope
  Scope1 : Scope
  Sum : Sum  Inputs=+++
  req : Outport
  wires:
  Sum/1 -> Scope/1, req/1
  p_cond/1 -> Scope1/1, Relay Level 3/1(in), Relay Level 2/1(in), Relay Level 1/1(in)
  Relay Level 3/1(out) -> Sum/1
  Relay Level 2/1(out) -> Sum/2
  Relay Level 1/1(out) -> Sum/3
  1-D Lookup Table/1 -> Relay Level 3/3(low), Bias/1
  Bias/1 -> Relay Level 3/2(high)
  1-D Lookup Table1/1 -> Relay Level 2/3(low), Bias1/1
  Bias1/1 -> Relay Level 2/2(high)
  1-D Lookup Table2/1 -> Relay Level 1/3(low), Bias2/1
  Bias2/1 -> Relay Level 1/2(high)
  T_env/1 -> 1-D Lookup Table/1, 1-D Lookup Table1/1, 1-D Lookup Table2/1

== system ElectricVehicleThermalManagementWithHeatPump/Controls/Fan Control/Inverter Requirement ==
  T_inverter : Inport
  Gain : Gain  Gain=1/3
  Relay Level 1 : Relay  OnSwitchValue=75  OffSwitchValue=65
  Relay Level 2 : Relay  OnSwitchValue=85  OffSwitchValue=76
  Relay Level 3 : Relay  OnSwitchValue=95  OffSwitchValue=86
  Sum : Sum  Inputs=+++
  cmd_fan : Outport
  wires:
  T_inverter/1 -> Relay Level 1/1, Relay Level 3/1, Relay Level 2/1
  Relay Level 2/1 -> Sum/2
  Relay Level 3/1 -> Sum/1
  Relay Level 1/1 -> Sum/3
  Sum/1 -> Gain/1
  Gain/1 -> cmd_fan/1

== system ElectricVehicleThermalManagementWithHeatPump/Controls/Fan Control/Motor Requirement ==
  T_motor : Inport
  1-D Lookup Table : Lookup_n-D  NumberOfTableDimensions=1  BreakpointsForDimension1=[-50 35 38 42 48 50 65 130]  IndexSearchMethod=Linear search  BeginIndexSearchUsingPreviousIndexResult=on  Table=[0 0 0.1 0.3 0.5 0.7 1 1]  InternalRulePriority=Speed  RndMeth=Simplest
  cmd_fan : Outport
  wires:
  T_motor/1 -> 1-D Lookup Table/1
  1-D Lookup Table/1 -> cmd_fan/1

== system ElectricVehicleThermalManagementWithHeatPump/Controls/Fan Control/Vehicle Speed Requirement ==
  v_vehicle : Inport
  Add : Sum  Inputs=++++
  Relay Level 1 : Relay  OnSwitchValue=20  OffSwitchValue=15
  Relay Level 2 : Relay  OnSwitchValue=60  OffSwitchValue=55
  Relay Level 3 : Relay  OnSwitchValue=75  OffSwitchValue=65
  Relay Level 4 : Relay  OnSwitchValue=90  OffSwitchValue=80
  req : Outport
  wires:
  Relay Level 4/1 -> Add/1
  Relay Level 3/1 -> Add/2
  Relay Level 2/1 -> Add/3
  Relay Level 1/1 -> Add/4
  Add/1 -> req/1
  v_vehicle/1 -> Relay Level 2/1, Relay Level 1/1, Relay Level 3/1, Relay Level 4/1

== system ElectricVehicleThermalManagementWithHeatPump/Controls/Thermal Mode/Mode Selection ==
  note: 0 = Off
      |
      | 1 = Cold loop
      |
      | 2 = Heat pump
  T_env : Inport
  Constant : Constant
  Constant1 : Constant  Value=0
  Constant2 : Constant  Value=2
  Switch : Switch  Criteria=u2 > Threshold  Threshold=19  SaturateOnIntegerOverflow=off  InputSameDT=off
  Switch1 : Switch  Threshold=21  SaturateOnIntegerOverflow=off  InputSameDT=off
  setpoint : Outport
  wires:
  T_env/1 -> Switch/2, Switch1/2
  Switch/1 -> setpoint/1
  Switch1/1 -> Switch/1
  Constant/1 -> Switch1/1
  Constant1/1 -> Switch1/3
  Constant2/1 -> Switch/3

== system ElectricVehicleThermalManagementWithHeatPump/Controls/Thermal Mode/Mode Transition ==
  note: 0 = Off
      |
      | 1 = Cold loop
      |
      | 2 = Heat pump
  setpoint : Inport
  rpm_comp : Inport  Port=2
  Memory : Memory
  Switch : Switch  Criteria=u2 > Threshold  SaturateOnIntegerOverflow=off  InputSameDT=off
  Transition from off to operating : Subsystem
  Transition from operating to off : Subsystem
  thermal_mode : Outport
  wires:
  setpoint/1 -> Transition from operating to off/2(setpoint), Transition from off to operating/1(setpoint)
  Transition from operating to off/1(mode) -> Switch/1
  Transition from off to operating/1(mode) -> Switch/3
  Memory/1 -> Transition from operating to off/1(current), Switch/2
  Switch/1 -> Memory/1, thermal_mode/1
  rpm_comp/1 -> Transition from off to operating/2(rpm_comp)

== system ElectricVehicleThermalManagementWithHeatPump/Controls/Valves Control/Chiller Expansion Valve ==
  thermal_mode : Inport
  T_coolant_battery_in : Inport  Port=2
  Constant : Constant  Value=0
  Constant1 : Constant  Value=0
  Multiport Switch : MultiPortSwitch  DataPortOrder=Zero-based contiguous  zeroidx=on  SaturateOnIntegerOverflow=off  InputSameDT=off
  Relay : Relay  OnSwitchValue=35  OffSwitchValue=25  OnOutputValue=0.024
  Scope : Scope
  Scope1 : Scope
  Transfer Fcn : TransferFcn  Denominator=[30 1]
  cmd_exv_chiller : Outport
  wires:
  thermal_mode/1 -> Multiport Switch/1
  Multiport Switch/1 -> cmd_exv_chiller/1
  Constant/1 -> Multiport Switch/2
  Constant1/1 -> Multiport Switch/4
  Transfer Fcn/1 -> Scope1/1, Multiport Switch/3
  Relay/1 -> Scope/1, Transfer Fcn/1
  T_coolant_battery_in/1 -> Relay/1

== system ElectricVehicleThermalManagementWithHeatPump/Controls/Valves Control/Evaporator Expansion Valve ==
  thermal_mode : Inport
  T_env : Inport  Port=2
  1-D Lookup Table : Lookup_n-D  NumberOfTableDimensions=1  BreakpointsForDimension1=[20 40]  BeginIndexSearchUsingPreviousIndexResult=on  Table=[0.006 0.009]  ExtrapMethod=Clip  InternalRulePriority=Speed  RndMeth=Simplest
  Constant : Constant  Value=0
  Constant1 : Constant  Value=0
  Multiport Switch : MultiPortSwitch  DataPortOrder=Zero-based contiguous  zeroidx=on  SaturateOnIntegerOverflow=off  InputSameDT=off
  cmd_exv_evap : Outport
  wires:
  thermal_mode/1 -> Multiport Switch/1
  Multiport Switch/1 -> cmd_exv_evap/1
  Constant/1 -> Multiport Switch/2
  Constant1/1 -> Multiport Switch/4
  1-D Lookup Table/1 -> Multiport Switch/3
  T_env/1 -> 1-D Lookup Table/1

== system ElectricVehicleThermalManagementWithHeatPump/Controls/Valves Control/Heat Pump Expansion Valve ==
  thermal_mode : Inport
  T_env : Inport  Port=2
  1-D Lookup Table : Lookup_n-D  NumberOfTableDimensions=1  BreakpointsForDimension1=[-10 0]  BeginIndexSearchUsingPreviousIndexResult=on  Table=[0.007 0.006]  ExtrapMethod=Clip  InternalRulePriority=Speed  RndMeth=Simplest
  Constant : Constant  Value=0
  Constant1 : Constant
  Multiport Switch : MultiPortSwitch  DataPortOrder=Zero-based contiguous  zeroidx=on  SaturateOnIntegerOverflow=off  InputSameDT=off
  Scope : Scope
  Scope1 : Scope
  cmd_exv_heatpump : Outport
  wires:
  thermal_mode/1 -> Scope1/1, Multiport Switch/1
  Multiport Switch/1 -> Scope/1, cmd_exv_heatpump/1
  Constant/1 -> Multiport Switch/2
  Constant1/1 -> Multiport Switch/3
  1-D Lookup Table/1 -> Multiport Switch/4
  T_env/1 -> 1-D Lookup Table/1

== system ElectricVehicleThermalManagementWithHeatPump/Controls/Valves Control/Radiator 3-Way Valve ==
  thermal_mode : Inport
  T_coolant_inverter_out : Inport  Port=2
  Constant : Constant  Value=0
  Memory : Memory
  Multiport Switch : MultiPortSwitch  DataPortOrder=Zero-based contiguous  zeroidx=on  SaturateOnIntegerOverflow=off  InputSameDT=off
  Relay : Relay  OnSwitchValue=50  OffSwitchValue=25  OnOutputValue=0  OffOutputValue=1
  Scope : Scope
  Scope1 : Scope
  cmd_rad_bypass : Outport
  wires:
  thermal_mode/1 -> Multiport Switch/1
  Relay/1 -> Scope1/1, Multiport Switch/4
  Constant/1 -> Multiport Switch/3
  Memory/1 -> Multiport Switch/2
  T_coolant_inverter_out/1 -> Scope/1, Relay/1
  Multiport Switch/1 -> Memory/1, cmd_rad_bypass/1

== system ElectricVehicleThermalManagementWithHeatPump/Controls/Valves Control/Refrigerant and Air 3-Way Valve ==
  thermal_mode : Inport
  Constant : Constant  Value=0
  Constant1 : Constant
  Memory : Memory
  Multiport Switch : MultiPortSwitch  DataPortOrder=Zero-based contiguous  zeroidx=on  SaturateOnIntegerOverflow=off  InputSameDT=off
  Scope : Scope
  Scope1 : Scope
  cmd_refrig_bypass : Outport
  cmd_blend_air : Outport  Port=2
  wires:
  thermal_mode/1 -> Scope/1, Multiport Switch/1
  Constant1/1 -> Multiport Switch/4
  Constant/1 -> Multiport Switch/3
  Multiport Switch/1 -> Scope1/1, cmd_blend_air/1, Memory/1, cmd_refrig_bypass/1
  Memory/1 -> Multiport Switch/2

== system ElectricVehicleThermalManagementWithHeatPump/Scenario/Power Demand/Derivative ==
  V : Inport
  Gain : Gain  Gain=1/tau
  Integrator : Integrator
  Sum : Sum  Inputs=|+-
  A : Outport
  wires:
  V/1 -> Sum/1
  Sum/1 -> Gain/1
  Gain/1 -> Integrator/1, A/1
  Integrator/1 -> Sum/2

== system ElectricVehicleThermalManagementWithHeatPump/Controls/Fan Control/Condenser Requirement/Relay Level 1 ==
  in : Inport
  high : Inport  Port=2
  low : Inport  Port=3
  Data Type Conversion : DataTypeConversion  SaturateOnIntegerOverflow=off  RndMeth=Floor
  Relational Operator : RelationalOperator  OutDataTypeStr=boolean  RndMeth=Simplest  InputSameDT=off
  Relational Operator1 : RelationalOperator  Operator=>  OutDataTypeStr=boolean  RndMeth=Simplest  InputSameDT=off
  Relay : Relay  OnSwitchValue=1.5  OffSwitchValue=0.5
  Sum : Sum  Inputs=|++
  out : Outport
  wires:
  Sum/1 -> Data Type Conversion/1
  Data Type Conversion/1 -> Relay/1
  Relational Operator1/1 -> Sum/2
  Relational Operator/1 -> Sum/1
  Relay/1 -> out/1
  low/1 -> Relational Operator1/2
  high/1 -> Relational Operator/2
  in/1 -> Relational Operator/1, Relational Operator1/1

== system ElectricVehicleThermalManagementWithHeatPump/Controls/Fan Control/Condenser Requirement/Relay Level 2 ==
  in : Inport
  high : Inport  Port=2
  low : Inport  Port=3
  Data Type Conversion : DataTypeConversion  SaturateOnIntegerOverflow=off  RndMeth=Floor
  Relational Operator : RelationalOperator  OutDataTypeStr=boolean  RndMeth=Simplest  InputSameDT=off
  Relational Operator1 : RelationalOperator  Operator=>  OutDataTypeStr=boolean  RndMeth=Simplest  InputSameDT=off
  Relay : Relay  OnSwitchValue=1.5  OffSwitchValue=0.5
  Sum : Sum  Inputs=|++
  out : Outport
  wires:
  Sum/1 -> Data Type Conversion/1
  Data Type Conversion/1 -> Relay/1
  Relational Operator1/1 -> Sum/2
  Relational Operator/1 -> Sum/1
  Relay/1 -> out/1
  low/1 -> Relational Operator1/2
  high/1 -> Relational Operator/2
  in/1 -> Relational Operator/1, Relational Operator1/1

== system ElectricVehicleThermalManagementWithHeatPump/Controls/Fan Control/Condenser Requirement/Relay Level 3 ==
  in : Inport
  high : Inport  Port=2
  low : Inport  Port=3
  Data Type Conversion : DataTypeConversion  SaturateOnIntegerOverflow=off  RndMeth=Floor
  Relational Operator : RelationalOperator  OutDataTypeStr=boolean  RndMeth=Simplest  InputSameDT=off
  Relational Operator1 : RelationalOperator  Operator=>  OutDataTypeStr=boolean  RndMeth=Simplest  InputSameDT=off
  Relay : Relay  OnSwitchValue=1.5  OffSwitchValue=0.5
  Sum : Sum  Inputs=|++
  out : Outport
  wires:
  Sum/1 -> Data Type Conversion/1
  Data Type Conversion/1 -> Relay/1
  Relational Operator1/1 -> Sum/2
  Relational Operator/1 -> Sum/1
  Relay/1 -> out/1
  low/1 -> Relational Operator1/2
  high/1 -> Relational Operator/2
  in/1 -> Relational Operator/1, Relational Operator1/1

== system ElectricVehicleThermalManagementWithHeatPump/Controls/Thermal Mode/Mode Transition/Transition from off to operating ==
  setpoint : Inport
  rpm_comp : Inport  Port=2
  Constant : Constant  Value=0
  Switch : Switch  Criteria=u2 > Threshold  Threshold=10  SaturateOnIntegerOverflow=off  InputSameDT=off
  mode : Outport
  wires:
  rpm_comp/1 -> Switch/2
  Switch/1 -> mode/1
  Constant/1 -> Switch/1
  setpoint/1 -> Switch/3
